simulink model "ASM_Traffic_A11"  (R2026a)
settings: Solver=ode1  StartTime=SIM.tstart.v  StopTime=SIM.tend.v  FixedStep=SIM.StepSize.v
PostLoadFcn:
  | if any(exist('dsrtsu_mdlpostloadfcn', 'file') ~= 0), dsrtsu_mdlpostloadfcn('Execute', bdroot); end
  | try, asm_mdl_postloadfcn(bdroot, 'UpdateModel', 3600); catch, disp(lasterr); end,
InitFcn:
  | , if any(exist('rtifpga_mdlclblib', 'file') ~= 0), rtifpga_mdlclblib('Init', bdroot); end,
  | , if any(exist('dsmpb_private', 'file') ~= 0), dsmpb_private('dsmpb_mdlclblib', 'Init', bdroot); end,
undefined symbols (not defined in the file): _to_, a0b2, ASM_BrakeHydraulics_DemoSystems, ASM_VehicleDynamics_DemoSystems, b98103fe8ad365046cd0, BrakeCircuit, controllerConfig, CPT, Crankshaft, DiscIntNeverNeededParam, dsmsi, FinalDriveAssembly, instance, MDL, ModeSignals, mu, Pos_BrakePedal_Maneuver, rad, RefSignals, s_to_rpm, SIM, SoftECU, Suspension, Tire, Transmission
libraries: ASM_Traffic_lib x135, simulink x98, ASM_Utils_lib x77, ASM_VehicleDynamics_lib x70, ASM_Environment_lib x22, dsmpblib x20, dsmsilib x15, MDLD_Utils_lib x10, ASM_BrakeHydraulics_lib x3, sl_discontinuities x2
(part 16 of 63)

== system ASM_Traffic_A11/VehicleDynamics/Plant/Sw_Plant_Signals ==
  PlantModel_Signals : Inport
  ExternalPlant_Signals : Inport  Port=2
  Angle_Gamma_FL_Wheel[deg] : Subsystem
  Bus Creator : BusCreator  Inputs=3
  Bus Creator1 : BusCreator  Inputs=2
  Bus Creator2 : BusCreator  Inputs=1
  Bus Creator3 : BusCreator  Inputs=2
  Bus Selector : BusSelector  OutputSignals=Steering.Displ_Steering[m],Steering.Displ_Steering_dt[m|s],RollerDyno.Angle_Gamma_FL_Wheel[deg],RollerDyno.omega_Wheel[rad|s]
  Bus Selector1 : BusSelector  OutputSignals=ExternalPlant.EPSMotor.Angle_EPSMotor[rad],ExternalPlant.EPSMotor.Angle_dt_EPSMotor[rad|s],ExternalPlant.Steering.Displ_Steering[m],ExternalPlant.Steering.Displ_Steering_dt[m|s],ExternalPlant.RollerDyno.Angle_Gamma_FL_Wheel[deg],ExternalPlant.RollerDyno.omega_Wheel[FL;FR;RL;RR][rad|s]
  Demux : Demux  Outputs=2
  Displ_SteeringRod[Displ;Displ_dt][m;m|s] : Subsystem
  EPSMotorStates_External[Angle;Angle_dt][rad;rad|s] : Subsystem
  EPS_External[Angle;Angle_dt][rad;rad|s]1 : Constant  Value=[0;0]
  Mux1 : Mux  Inputs=2
  Mux2 : Mux  Inputs=2
  Mux3 : Mux  Inputs=2
  omega_Wheel[FL;FR;RL;RR][rad|s] : Subsystem
  Plant_Signals : Outport  VectorParamsAs1DForOutWhenUnconnected=off
  wires:
  Demux/1 -> Bus Creator1/1  "Displ_Steering[m]"
  Demux/2 -> Bus Creator1/2  "Displ_Steering_dt[m|s]"
  Displ_SteeringRod[Displ;Displ_dt][m;m|s]/1(Displ_SteeringRod[Displ;Displ_dt][m;m|s]) -> Demux/1  "Displ_SteeringRod[Displ;Displ_dt][m;m|s]"
  EPS_External[Angle;Angle_dt][rad;rad|s]1/1 -> EPSMotorStates_External[Angle;Angle_dt][rad;rad|s]/1(SoftECU)
  Mux3/1 -> Displ_SteeringRod[Displ;Displ_dt][m;m|s]/1(SoftECU)
  Bus Selector/2 -> Mux3/2  "<Displ_Steering_dt[m|s]>"
  Bus Selector/1 -> Mux3/1  "<Displ_Steering[m]>"
  Mux1/1 -> EPSMotorStates_External[Angle;Angle_dt][rad;rad|s]/2(RealECU)
  Mux2/1 -> Displ_SteeringRod[Displ;Displ_dt][m;m|s]/2(RealECU)
  Bus Selector1/4 -> Mux2/2  "<Displ_Steering_dt[m|s]>"
  Bus Selector1/3 -> Mux2/1  "<Displ_Steering[m]>"
  Bus Selector1/2 -> Mux1/2  "<Angle_dt_EPSMotor[rad|s]>"
  Bus Selector1/1 -> Mux1/1  "<Angle_EPSMotor[rad]>"
  EPSMotorStates_External[Angle;Angle_dt][rad;rad|s]/1(EPSMotorStates_External[Angle;Angle_dt][rad;rad|s]) -> Bus Creator2/1  "EPSMotorStates_External[Angle;Angle_dt][rad;rad|s]"
  Bus Creator2/1 -> Bus Creator/1  "EPSMotor"
  Bus Creator1/1 -> Bus Creator/2  "Steering"
  Bus Creator/1 -> Plant_Signals/1  "ActivePlant"
  ExternalPlant_Signals/1 -> Bus Selector1/1
  PlantModel_Signals/1 -> Bus Selector/1
  Bus Selector1/5 -> Angle_Gamma_FL_Wheel[deg]/2(RealECU)  "<Angle_Gamma_FL_Wheel[deg]>"
  Bus Selector1/6 -> omega_Wheel[FL;FR;RL;RR][rad|s]/2(RealECU)  "<omega_Wheel[FL;FR;RL;RR][rad|s]>"
  omega_Wheel[FL;FR;RL;RR][rad|s]/1(omega_Wheel[FL;FR;RL;RR][rad|s]) -> Bus Creator3/2  "omega_Wheel[FL;FR;RL;RR][rad|s]"
  Angle_Gamma_FL_Wheel[deg]/1(Angle_Gamma_FL_Wheel[deg]) -> Bus Creator3/1  "Angle_Gamma_FL_Wheel[deg]"
  Bus Creator3/1 -> Bus Creator/3  "RollerDyno"
  Bus Selector/3 -> Angle_Gamma_FL_Wheel[deg]/1(SoftECU)  "<Angle_Gamma_FL_Wheel[deg]>"
  Bus Selector/4 -> omega_Wheel[FL;FR;RL;RR][rad|s]/1(SoftECU)  "<omega_Wheel[rad|s]>"

== system ASM_Traffic_A11/VehicleDynamics/Plant/UserInterface ==
  note: Vehicle Dynamics
  In : Inport
  ASMSignalBus_Plant : Subsystem
  DISP_Plant : Subsystem
  PAR_Plant : Subsystem
  Out : Outport  VectorParamsAs1DForOutWhenUnconnected=off
  wires:
  PAR_Plant/1(Out) -> Out/1
  In/1 -> ASMSignalBus_Plant/1(In), DISP_Plant/1(In)

== system ASM_Traffic_A11/VehicleDynamics/Plant/VehicleDynamics ==
  UserInterface : Inport
  Interface_In : Inport  Port=2
  Control : Inport  Port=3
  Plant_Signals : Inport  Port=4
  AERODYNAMICS : ASM_VehicleDynamics_lib/VehicleDynamics/Aerodynamics/AERODYNAMICS  Tag=ASM_SUBCOMPONENT  Map_C_x=MDL.VehicleDynamics.Aerodynamics.Map_C_x  Map_C_y=MDL.VehicleDynamics.Aerodynamics.Map_C_y  Map_C_z=MDL.VehicleDynamics.Aerodynamics.Map_C_z  Map_C_M_x=MDL.VehicleDynamics.Aerodynamics.Map_C_M_x  Map_C_M_y=MDL.VehicleDynamics.Aerodynamics.Map_C_M_y  Map_C_M_z=MDL.VehicleDynamics.Aerodynamics.Map_C_M_z  Const_A_x=MDL.VehicleDynamics.Aerodynamics.Const_A_x  Const_PosVec_VtoRefAero=MDL.VehicleDynamics.Aerodynamics.Const_PosVec_RefAero_CoorSysV  Const_Char_Length=MDL.VehicleDynamics.Aerodynamics.Const_Char_Length  Const_Dens_Air=MDL.VehicleDynamics.Aerodynamics.Const_Dens_Air  ASMProperties=struct('Name','AERODYNAMICS','Version','5.0','Library','ASM_VehicleDynamics_lib')  ASMInstanceName=aerodynamics  ASMInstanceID=1
  ASMSignalCollector : Subsystem
  Brake : Subsystem
  Bus Selector1 : BusSelector  OutputSignals=ExternalModel.Sw_Tire_Parameter_Set_CP[FL;FR;RL;RR][1|2|3|4],ExternalModel.Fric_Coeff_CP[FL;FR;RL;RR][],ExternalModel.Pos_z_CP[FL;FR;RL;RR][m],ExternalModel.UnitVec_z_CP[FL;FR;RL;RR][x;y;z],ExternalModel.Pos_Vehicle_Init_CoorSys_E[x;y;z][m],ExternalModel.Angle_Vehicle_Init_CoorSys_E[x;y;z][rad],ExternalModel.Reset_VehicleStates[0|1],ExternalModel.Keep_VehiclePosition[0|1],ExternalModel.Pos_BrakePedal[%],ExternalModel.Angle_SteeringWheel[deg],ExternalModel.v_Wind_Coor_Sys_E[x;y;z][m|s],ExternalModel.p_Ambient[Pa],ExternalModel.Sw_ParkingBrake[0Off|1On],ExternalModel.T_Ambient[degC],ExternalModel.Pos_AccPedal[%],ExternalModel.q_dt_Vehicle_Init[6x1],ExternalModel.Trq_Driver_External[Nm],ExternalModel.Sw_SteeringMode[1Angle|2Trq],ExternalModel.Sw_Steering_Mode[1Manual|2ManSched],ExternalModel.Const_Steering_Mode_Manual[1Angle|2Trq]
  Bus Selector10 : BusSelector  OutputSignals=ExternalModel.Q_Articulated_T[6x1],ExternalModel.Trq_Hitch_CoorSys_V[x;y;z][Nm],ExternalModel.M_Articulated_T[1x36]
  Bus Selector2 : BusSelector  OutputSignals=w_Rel_FL_Wheel_dDispl_SteeringRod_dt[x;y;z][rad|m],w_Rel_FR_Wheel_dDispl_SteeringRod_dt[x;y;z][rad|m]  OutputAsBus=on
  Bus Selector3 : BusSelector  OutputSignals=Pos_FL_Wheel_dDispl_SteeringRod[x;y;z][],Pos_FR_Wheel_dDispl_SteeringRod[x;y;z][]  OutputAsBus=on
  Bus Selector4 : BusSelector  OutputSignals=ECU_Steering.Trq_PowerSteering[Nm]
  Bus Selector6 : BusSelector  OutputSignals=ECU_Brake.ECU_Mode.ECU_ESP_Mode[0None|1ABS|2ESP|3ASR],ECU_Brake.Valves.Ctrl_InletValve_FL[0_1],ECU_Brake.Valves.Ctrl_InletValve_FR[0_1],ECU_Brake.Valves.Ctrl_InletValve_RL[0_1],ECU_Brake.Valves.Ctrl_InletValve_RR[0_1],ECU_Brake.Valves.Ctrl_OutletValve_FL[0_1],ECU_Brake.Valves.Ctrl_OutletValve_FR[0_1],ECU_Brake.Valves.Ctrl_OutletValve_RL[0_1],ECU_Brake.Valves.Ctrl_OutletValve_RR[0_1],ECU_Brake.Valves.Ctrl_PreChargeValve_1[0_1],ECU_Brake.Valves.Ctrl_PreChargeValve_2[0_1],ECU_Brake.Valves.Ctrl_ChangeOverValve_1[0_1],ECU_Brake.Valves.Ctrl_ChangeOverValve_2[0_1],ECU_Brake.Valves.Ctrl_HydPump[0_1],ECU_Brake.DesiredPressure.Enable_p_Brake_Desired[0|1],ECU_Brake.DesiredPressure.p_Brake_Desired[bar]  OutputAsBus=on
  Bus Selector7 : BusSelector  OutputSignals=Tire.Tire.Sw_r_Tire[1:intern;2:extern],Tire.Tire.r_Tire_extern[m],Suspension.Suspension_Init.q_dt_Wheel_Init[:],Suspension.Suspension_Init.q_Wheel_Init[:],BrakeHydraulics.Sw_DistributionPattern_[1X|2II],Suspension.Sw_Rotation[1Cardan|2ToeCamberCaster]
  Bus Selector8 : BusSelector  OutputSignals=Steering.Displ_Steering_dt[m|s],Steering.Displ_Steering[m],RollerDyno.omega_Wheel[FL;FR;RL;RR][rad|s],EPSMotor.EPSMotorStates_External[Angle;Angle_dt][rad;rad|s],RollerDyno.Angle_Gamma_FL_Wheel[deg]
  Bus Selector9 : BusSelector  OutputSignals=ExternalModel.Trq_Shaft[FL;FR;RL;RR][Nm]
  CommonVehicleParameters : Subsystem
      settings: CopyFcn=|
      | try
      |  set_param(gcb,'LinkStatus', 'none')
      | catch
      | end
      mask Display: disp('Common vehicle parameters')
  Constant : Constant  Value=0
  DerivativeAddition : Subsystem
  Exchangeable_Plant_Signals : Subsystem
  Goto Tag Visibility : GotoTagVisibility  GotoTag=ASMBUS_VehicleDynamics_Tire
  Goto Tag Visibility1 : GotoTagVisibility  GotoTag=ASMBUS_VehicleDynamics_Aerodynamics
  Goto Tag Visibility10 : GotoTagVisibility  GotoTag=TAG_VehicleDynamics_Inertia_y_RL_Wheel
  Goto Tag Visibility11 : GotoTagVisibility  GotoTag=TAG_VehicleDynamics_Inertia_y_RR_Wheel
  Goto Tag Visibility12 : GotoTagVisibility  GotoTag=TAG_VehicleDynamics_Coef_DynamicBrakeTrq
  Goto Tag Visibility13 : GotoTagVisibility  GotoTag=TAG_VehicleDynamics_m_RR_Wheel
  Goto Tag Visibility14 : GotoTagVisibility  GotoTag=TAG_VehicleDynamics_Inertia_FL_Wheel
  Goto Tag Visibility15 : GotoTagVisibility  GotoTag=TAG_VehicleDynamics_Inertia_FR_Wheel
  Goto Tag Visibility16 : GotoTagVisibility  GotoTag=TAG_VehicleDynamics_Inertia_RL_Wheel
  Goto Tag Visibility17 : GotoTagVisibility  GotoTag=TAG_VehicleDynamics_Inertia_RR_Wheel
  Goto Tag Visibility18 : GotoTagVisibility  GotoTag=TAG_VehicleDynamics_Inertia_y_FL_Wheel
  Goto Tag Visibility19 : GotoTagVisibility  GotoTag=TAG_VehicleDynamics_Inertia_y_FR_Wheel
  Goto Tag Visibility2 : GotoTagVisibility  GotoTag=ASMBUS_VehicleDynamics_VehicleMovement
  Goto Tag Visibility20 : GotoTagVisibility  GotoTag=ASMBUS_VehicleDynamics_Steering_Rod_Back_Calc
  Goto Tag Visibility3 : GotoTagVisibility  GotoTag=ASMBUS_VehicleDynamics_WheelSpeed
  Goto Tag Visibility4 : GotoTagVisibility  GotoTag=ASMBUS_VehicleDynamics_Suspension
  Goto Tag Visibility5 : GotoTagVisibility  GotoTag=ASMBUS_VehicleDynamics_Brake
  Goto Tag Visibility6 : GotoTagVisibility  GotoTag=ASMBUS_VehicleDynamics_Steering
  Goto Tag Visibility7 : GotoTagVisibility  GotoTag=TAG_VehicleDynamics_m_FL_Wheel
  Goto Tag Visibility8 : GotoTagVisibility  GotoTag=TAG_VehicleDynamics_m_FR_Wheel
  Goto Tag Visibility9 : GotoTagVisibility  GotoTag=TAG_VehicleDynamics_m_RL_Wheel
  Hitch_Vehicle : Subsystem
      settings: CopyFcn=|
      | try
      |  set_param(gcb,'LinkStatus', 'none')
      | catch
      | end
  ModelDesk_MC_ID_VehicleDynamics : ASM_Utils_lib/ModelDeskInterface/ModelDesk_MC  Tag=ASM_MAINCOMPONENT  Editable=off  MainComponent=VehicleDynamics
  Multiport Switch : MultiPortSwitch  Inputs=2  SaturateOnIntegerOverflow=off  InputSameDT=off
  OR : Subsystem
  STEERING_3DOF_VARIABLE_RATIO : ASM_VehicleDynamics_lib/VehicleDynamics/Steering/STEERING_3DOF_VARIABLE_RATIO  Tag=ASM_SUBCOMPONENT  SW_EPSLocation=MDL.VehicleDynamics.Steering3DOF.SW_EPSLocation  SW_EPSSimulation=MDL.VehicleDynamics.Steering3DOF.SW_EPSSimulation  SW_ExternalEPSOutput=MDL.VehicleDynamics.Steering3DOF.SW_ExternalEPSOutput  SW_LocationColumnStiffness=MDL.VehicleDynamics.Steering3DOF.SW_LocationColumnStiffness  SW_DriverHand=MDL.VehicleDynamics.Steering3DOF.SW_DriverHand  Map_i_Steering=MDL.VehicleDynamics.Steering3DOF.Map_i_Steering  Const_i_EPSSteeringColumn=MDL.VehicleDynamics.Steering3DOF.Const_i_EPSSteeringColumn  Const_i_EPSSteeringRod=MDL.VehicleDynamics.Steering3DOF.Const_i_EPSSteeringRod  Const_Angle_Max_SteeringWheel=MDL.VehicleDynamics.Steering3DOF.Const_Angle_Max_SteeringWheel  Const_CardanAngle_UpperJoint=MDL.VehicleDynamics.Steering3DOF.Const_CardanAngle_UpperJoint  Const_CardanAngle_LowerJoint=MDL.VehicleDynamics.Steering3DOF.Const_CardanAngle_LowerJoint  Const_AngleOffsetCardanJoints=MDL.VehicleDynamics.Steering3DOF.Const_InitialAngle_LowerCardanJoint  Const_InitialAngle_UpperCardanJoint=MDL.VehicleDynamics.Steering3DOF.Const_InitialAngle_UpperCardanJoint  Const_MaxTorque_Driver=MDL.VehicleDynamics.Steering3DOF.Const_MaxTorque_Driver  Const_Inertia_SteeringWheel=MDL.VehicleDynamics.Steering3DOF.Const_Inertia_SteeringWheel  Const_Inertia_LowerSteeringColumn=MDL.VehicleDynamics.Steering3DOF.Const_Inertia_LowerSteeringColumn  SW_SteeringColumn_Stiffness=MDL.VehicleDynamics.Steering3DOF.SW_SteeringColumn_Stiffness  Map_TrqSpring_SteeringColumn=MDL.VehicleDynamics.Steering3DOF.Map_TrqSpring_SteeringColumn  Const_Stiffness_SteeringColumn=MDL.VehicleDynamics.Steering3DOF.Const_Stiffness_SteeringColumn  Const_Damping_SteeringColumn=MDL.VehicleDynamics.Steering3DOF.Const_Damping_SteeringColumn  Const_Time_SteeringWheel=MDL.VehicleDynamics.Steering3DOF.Const_Time_SteeringWheel  Const_Stiffness_DriverHand=MDL.VehicleDynamics.Steering3DOF.Const_Stiffness_DriverHand  Const_Damping_DriverHand=MDL.VehicleDynamics.Steering3DOF.Const_Damping_DriverHand  Const_Inertia_EPS=MDL.VehicleDynamics.Steering3DOF.Const_Inertia_EPS  Const_Stiffness_EPS=MDL.VehicleDynamics.Steering3DOF.Const_Stiffness_EPS  Const_Damping_EPS=MDL.VehicleDynamics.Steering3DOF.Const_Damping_EPS  Const_Damping_LowerSteeringColumn=MDL.VehicleDynamics.Steering3DOF.Const_Damping_LowerSteeringColumn  SW_SF_SteeringWheel=MDL.VehicleDynamics.Steering3DOF.SpringFriction.SW_SF_SteeringWheel  Const_Stiffness_SF_SteeringWheel=MDL.VehicleDynamics.Steering3DOF.SpringFriction.Const_Stiffness_SF_SteeringWheel  Const_LimitingTorque_SF_SteeringWheel=MDL.VehicleDynamics.Steering3DOF.SpringFriction.Const_LimitingTorque_SF_SteeringWheel  SW_ESF_SteeringWheel=MDL.VehicleDynamics.Steering3DOF.ExponentialSpringFriction.SW_ESF_SteeringWheel  Const_Stiffness_ESF_SteeringWheel=MDL.VehicleDynamics.Steering3DOF.ExponentialSpringFriction.Const_Stiffness_ESF_SteeringWheel  Const_LimitingTorque_ESF_SteeringWheel=MDL.VehicleDynamics.Steering3DOF.ExponentialSpringFriction.Const_LimitingTorque_ESF_SteeringWheel  SW_CF_SteeringRod=MDL.VehicleDynamics.Steering3DOF.CoulombFriction.SW_CF_SteeringRod  Const_LimitingForce_CF_SteeringRod=MDL.VehicleDynamics.Steering3DOF.CoulombFriction.Const_LimitingForce_CF_SteeringRod  Const_Damping_CF_SteeringRod=MDL.VehicleDynamics.Steering3DOF.CoulombFriction.Const_Damping_CF_SteeringRod  SW_MF_SteeringRod=MDL.VehicleDynamics.Steering3DOF.MaxwellFriction.SW_MF_SteeringRod  Const_Stiffness_MF_SteeringRod=MDL.VehicleDynamics.Steering3DOF.MaxwellFriction.Const_Stiffness_MF_SteeringRod  Const_LimitingForce_MF_SteeringRod=MDL.VehicleDynamics.Steering3DOF.MaxwellFriction.Const_LimitingForce_MF_SteeringRod  Const_Damping_MF_SteeringRod=MDL.VehicleDynamics.Steering3DOF.MaxwellFriction.Const_Damping_MF_SteeringRod  SW_SF_SteeringRod=MDL.VehicleDynamics.Steering3DOF.SpringFriction.SW_SF_SteeringRod  Const_Stiffness_SF_SteeringRod=MDL.VehicleDynamics.Steering3DOF.SpringFriction.Const_Stiffness_SF_SteeringRod  Const_LimitingForce_SF_SteeringRod=MDL.VehicleDynamics.Steering3DOF.SpringFriction.Const_LimitingForce_SF_SteeringRod  SW_ESF_SteeringRod=MDL.VehicleDynamics.Steering3DOF.ExponentialSpringFriction.SW_ESF_SteeringRod  Const_Stiffness_ESF_SteeringRod=MDL.VehicleDynamics.Steering3DOF.ExponentialSpringFriction.Const_Stiffness_ESF_SteeringRod  Const_LimitingForce_ESF_SteeringRod=MDL.VehicleDynamics.Steering3DOF.ExponentialSpringFriction.Const_LimitingForce_ESF_SteeringRod  StepSize=SIM.StepSize  ASMProperties=struct('Name','STEERING_3DOF_VARIABLE_RATIO','Version','10.0','Library','ASM_VehicleDynamics_lib')  ASMInstanceName=steering_3dof_variable_ratio  ASMInstanceID=1
  STEERING_ROD_BACK_CALC : ASM_VehicleDynamics_lib/VehicleDynamics/STEERING_ROD_BACK_CALC  Tag=ASM_SUBCOMPONENT  Map_Displ_SteeringRod=MDL.VehicleDynamics.SteeringRodBackCalc.Map_Displ_SteeringRod  Sw_Backward_SteeringRod_Calc=MDL.VehicleDynamics.SteeringRodBackCalc.Sw_Backward_SteeringRod_Calc  Const_NaturalFrequency_Displ_SteeringRod=MDL.VehicleDynamics.SteeringRodBackCalc.Const_NaturalFrequency_Displ_SteeringRod  ASMProperties=struct('Name','STEERING_ROD_BACK_CALC','Version','1.0','Library','ASM_VehicleDynamics_lib')  ASMInstanceName=steering_rod_back_calc  ASMInstanceID=1
  SignalSpecification : SignalSpecification  Dimensions=4
  Suspension : Subsystem
  Terminator{,1..3} (4 alike) : Terminator
  Tire : Subsystem
  TireMapping_CP : Subsystem
      mask Display: disp('');
  VehicleInits : Subsystem
  VehicleMovement : Subsystem
  WHEEL_SPEED : ASM_VehicleDynamics_lib/VehicleDynamics/WheelSpeed/WHEEL_SPEED  Tag=ASM_SUBCOMPONENT  StepSize=SIM.StepSize  ASMProperties=struct('Name','WHEEL_SPEED','Version','11.0','Library','ASM_VehicleDynamics_lib')  ASMInstanceName=wheel_speed  ASMInstanceID=1
  "[1x36]to[6x6]" : Reshape  OutputDimensionality=Customize  OutputDimensions=[6,6]
  avoid_incomplete_trace2source : Subsystem
  avoid_incomplete_trace2source1 : Subsystem
  avoid_incomplete_trace2source2 : Subsystem
  ASMSignalBus : Outport  VectorParamsAs1DForOutWhenUnconnected=off
  PlantModel_Signals : Outport  Port=2  VectorParamsAs1DForOutWhenUnconnected=off
  tag scope: ASMBUS_VehicleDynamics_Aerodynamics=scoped, ASMBUS_VehicleDynamics_Brake=scoped, ASMBUS_VehicleDynamics_Steering=scoped, ASMBUS_VehicleDynamics_Steering_Rod_Back_Calc=scoped, ASMBUS_VehicleDynamics_Suspension=scoped, ASMBUS_VehicleDynamics_Tire=scoped, ASMBUS_VehicleDynamics_VehicleMovement=scoped, ASMBUS_VehicleDynamics_WheelSpeed=scoped
  wires:
  avoid_incomplete_trace2source2/1(Out1) -> WHEEL_SPEED/7
  Bus Selector8/3 -> avoid_incomplete_trace2source2/1(In1)  "<omega_Wheel[FL;FR;RL;RR][rad|s]>"
  avoid_incomplete_trace2source1/1(Out1) -> WHEEL_SPEED/5
  avoid_incomplete_trace2source/1(Out1) -> WHEEL_SPEED/1
  Tire/5(Trq_Tire_Wheel[FL,FR,RL,RR][Nm]) -> avoid_incomplete_trace2source/1(In1)
  Bus Selector8/5 -> STEERING_ROD_BACK_CALC/1  "<Angle_Gamma_FL_Wheel[deg]>"
  Interface_In/1 -> Bus Selector10/1, Bus Selector1/1, Bus Selector9/1
  Brake/1(ASMSignalBus) -> [ASMBUS_VehicleDynamics_Brake]
  AERODYNAMICS/1 -> [ASMBUS_VehicleDynamics_Aerodynamics]
  WHEEL_SPEED/1 -> [ASMBUS_VehicleDynamics_WheelSpeed]
  WHEEL_SPEED/3 -> VehicleMovement/6(w_Wheel[FL,FR,RL,RR][x;y;z][rad|s])
  Tire/3(Trq_Tire_CoorSys_V[FL,FR,RL,RR][x;y;z][Nm]) -> VehicleMovement/4(Trq_Tire_CoorSys_V[FL,FR,RL,RR][x;y;z][Nm]), STEERING_3DOF_VARIABLE_RATIO/4, Suspension/4(Trq_Tire[FL;FR;RL;RR][x;y;z][Nm])
  STEERING_3DOF_VARIABLE_RATIO/1 -> [ASMBUS_VehicleDynamics_Steering]
  Tire/2(F_Tire_CoorSys_V[FL,FR,RL,RR][x;y;z][N]) -> STEERING_3DOF_VARIABLE_RATIO/3, Suspension/3(F_Tire[FL;FR;RL;RR][x;y;z][N]), VehicleMovement/3(F_Tire_CoorSys_V[FL,FR,RL,RR][x;y;z][N])
  VehicleMovement/4(Pos_Wheels_CoorSys_E[FL,FR,RL,RR][x;y;z][m]) -> Tire/3(Pos_Wheels_CoorSys_E[FL,FR,RL,RR][x,y,z][m])
  VehicleMovement/5(v_Abs_WheelBody_CoorSys_V[FL,FR,RL,RR][x y z][m|s]) -> Tire/4(v_Abs_WheelBody_CoorSys_V[FL,FR,RL,RR][x;y;z][m|s])
  VehicleMovement/6(w_Abs_Wheel_CoorSys_V[FL,FR,RL,RR][x,y,z][rad|s]) -> Tire/5(w_Abs_Wheel_CoorSys_V[FL,FR,RL,RR][x,y,z][rad|s])
  VehicleMovement/3(RotationMatrix_V_to_E_T[3x3]) -> Tire/2(RotationMatrix_V_to_E_T[3x3]), AERODYNAMICS/1
  AERODYNAMICS/2 -> VehicleMovement/2(Trq_Aero_CoorSys_V[x;y;z][Nm])
  AERODYNAMICS/3 -> VehicleMovement/1(F_Aero_CoorSys_V[x;y;z][N])
  VehicleMovement/1(ASMSignalBus) -> [ASMBUS_VehicleDynamics_VehicleMovement]
  VehicleMovement/2(v_Abs_Vehicle_CoG[x;y;z][m|s]) -> AERODYNAMICS/2
  Brake/2(Trq_Brake[FL,FR,RL,RR][Nm]) -> WHEEL_SPEED/3
  Bus Selector1/7 -> Brake/1(Reset[]), STEERING_ROD_BACK_CALC/4, STEERING_3DOF_VARIABLE_RATIO/7, OR/2(In2), VehicleMovement/14(Reset[]), Suspension/6(Reset[]), avoid_incomplete_trace2source1/1(In1)  "<Reset_VehicleStates[0|1]>"
  Bus Selector1/9 -> Brake/2(Pos_BrakePedal[%])  "<Pos_BrakePedal[%]>"
  Bus Selector1/11 -> AERODYNAMICS/3  "<v_Wind_Coor_Sys_E[x;y;z][m|s]>"
  Suspension/1(ASMSignalBus) -> [ASMBUS_VehicleDynamics_Suspension]
  VehicleMovement/8(Trq_Gyroscopic[FL,FR,RL,RR][x;y;z][Nm]) -> STEERING_3DOF_VARIABLE_RATIO/9
  VehicleMovement/7(F_Gyroscopic[FL,FR,RL,RR][x;y;z][N]) -> STEERING_3DOF_VARIABLE_RATIO/8
  VehicleMovement/9(F_Gravitational[FL,FR,RL,RR][x;y;z][N]) -> STEERING_3DOF_VARIABLE_RATIO/10
  Suspension/10(UnitVec_y_Wheel_CoorSys_V[FL,FR,RL,RR][x;y;z]) -> Tire/1(UnitVec_y_Wheel_CoorSys_V[FL,FR,RL,RR][x;y;z]), WHEEL_SPEED/4
  Bus Selector6/1 -> Brake/3(IO_Signals)
  Bus Selector1/6 -> VehicleMovement/13(Angle_V_Init_CoorSys_E[x;y;z][rad])  "<Angle_Vehicle_Init_CoorSys_E[x;y;z][rad]>"
  Bus Selector1/5 -> VehicleMovement/12(Pos_Vehicle_Init_CoorSys_E[x;y;z][m])  "<Pos_Vehicle_Init_CoorSys_E[x;y;z][m]>"
  Tire/1(ASMSignalBus) -> [ASMBUS_VehicleDynamics_Tire]
  Tire/4(Stiffness_z_Tire[FL,FR,RL,RR][N|m]) -> VehicleMovement/5(Stiffness_z_Tire[FL,FR,RL,RR][N|m])
  Bus Selector9/1 -> SignalSpecification/1  "<Trq_Shaft[FL;FR;RL;RR][Nm]>"
  WHEEL_SPEED/4 -> Exchangeable_Plant_Signals/1(omega_Wheel[rad|s]), Tire/11(omega_Wheel[FL,FR,RL,RR][rad|s])
  WHEEL_SPEED/2 -> STEERING_3DOF_VARIABLE_RATIO/5, VehicleMovement/7(Trq_Shaft_CoorSys_V[FL,FR,RL,RR][x;y;z][Nm])
  Suspension/9(gF_Susp[q1_Front;q2_Front;q1_Rear;q2_Rear][]) -> VehicleMovement/8(gF_Susp[q1_Front;q2_Front;q1_Rear;q2_Rear][])
  Suspension/8(Pos_Wheels[FL,FR,RL,RR][x;y;z][m]) -> VehicleMovement/9(Pos_Wheel[FL,FR,RL,RR][x;y;z][m])
  Suspension/7(w_Rel_WheelBody[FL,FR,RL,RR][x;y;z][x;y;z][rad|s]) -> VehicleMovement/10(w_Rel_WheelBody[FL,FR,RL,RR][x y z][rad|s])
  Suspension/6(v_Rel_WheelBody[FL,FR,RL,RR][x;y;z][m|s]) -> VehicleMovement/11(v_Rel_WheelBody[FL,FR,RL,RR][x;y;z][m|s])
  VehicleMovement/10(q_Wheel_dt[q1_Front;q2_Front;q1_Rear;q2_Rear][]) -> Suspension/2(q_Wheel_dt[q1_Front;q2_Front;q1_Rear;q2_Rear][])
  VehicleMovement/11(q_Wheel[q1_Front;q2_Front;q1_Rear;q2_Rear][]) -> Suspension/1(q_Wheel[q1_Front;q2_Front;q1_Rear;q2_Rear][])
  Suspension/2(SuspensionKinematicRelations_Front) -> VehicleMovement/19(SuspensionKinematicsRelations_Front), Bus Selector3/1, Bus Selector2/1
  Suspension/3(SuspensionKinematicRelations_Rear) -> VehicleMovement/18(SuspensionKinematicsRelations_Rear)
  Suspension/4(gFront_dq_Front_dt[2x2][]) -> VehicleMovement/17(gFront_dq_Front_dt[2x2][])
  Suspension/5(gRear_dq_Rear_dt[2x2][]) -> VehicleMovement/16(gRear_dq_Rear_dt[2x2][])
  Bus Selector1/10 -> DerivativeAddition/1(Angle_SteeringWheel_Driver[deg])  "<Angle_SteeringWheel[deg]>"
  Bus Selector1/12 -> Brake/4(p_Ambient[Pa])  "<p_Ambient[Pa]>"
  SignalSpecification/1 -> WHEEL_SPEED/2
  Bus Selector1/13 -> Brake/5(Sw_ParkingBrake[0Off|1On])  "<Sw_ParkingBrake[0Off|1On]>"
  Hitch_Vehicle/1(F_External_CoorSys_V[x;y;z][N]) -> VehicleMovement/20(F_External_CoorSys_V[x,y,z][N])
  Hitch_Vehicle/2(Trq_External_CoorSys_V[x;y;z][Nm]) -> VehicleMovement/21(Trq_External_CoorSys_V[x,y,z][Nm])
  Hitch_Vehicle/3(Stabilization_F_External[3x6]) -> VehicleMovement/22(Stabilization_F_External[3X6])
  Hitch_Vehicle/4(Stabilization_Trq_External[3x6]) -> VehicleMovement/23(Stabilization_Trq_External[3X6])
  STEERING_3DOF_VARIABLE_RATIO/4 -> Terminator/1
  Bus Selector1/14 -> Brake/6(T_Ambient[degC])  "<T_Ambient[degC]>"
  Bus Selector1/15 -> Brake/7(Pos_AccPedal[%])  "<Pos_AccPedal[%]>"
  Bus Selector1/8 -> VehicleMovement/15(KeepVehiclePosition[0|1]), OR/1(In1)  "<Keep_VehiclePosition[0|1]>"
  OR/1(Out) -> Tire/10(Reset[])
  VehicleInits/1(omega_Wheel_Init[:][rad|s]) -> WHEEL_SPEED/6
  Bus Selector1/1 -> TireMapping_CP/1(Sw_Tire_Parameter_Set_CP[:][1|2|3|4])  "<Sw_Tire_Parameter_Set_CP[FL;FR;RL;RR][1|2|3|4]>"
  Bus Selector1/16 -> VehicleInits/1(q_dt_Vehicle_Init[6x1])  "<q_dt_Vehicle_Init[6x1]>"
  VehicleInits/3(q_Wheel_Init[:]) -> VehicleMovement/25(q_Wheel_Init[:])
  VehicleInits/2(q_dt_Init[:]) -> VehicleMovement/24(q_dt_Init[:])
  DerivativeAddition/1(SteeringWheel_Driver[Angle;Angle_dt][deg;deg|s]) -> STEERING_3DOF_VARIABLE_RATIO/6
  Bus Selector2/1 -> STEERING_3DOF_VARIABLE_RATIO/1
  Bus Selector3/1 -> STEERING_3DOF_VARIABLE_RATIO/2
  Bus Selector1/17 -> STEERING_3DOF_VARIABLE_RATIO/12  "<Trq_Driver_External[Nm]>"
  Bus Selector1/18 -> Multiport Switch/3  "<Sw_SteeringMode[1Angle|2Trq]>"
  Constant/1 -> Suspension/5(AirSuspensionSignals_In)
  Suspension/11(AirSuspensionSignals_Out) -> Terminator3/1
  Bus Selector1/19 -> Multiport Switch/1  "<Sw_Steering_Mode[1Manual|2ManSched]>"
  Bus Selector1/20 -> Multiport Switch/2  "<Const_Steering_Mode_Manual[1Angle|2Trq]>"
  Multiport Switch/1 -> STEERING_3DOF_VARIABLE_RATIO/13
  Control/1 -> Bus Selector6/1, Bus Selector4/1
  Bus Selector4/1 -> STEERING_3DOF_VARIABLE_RATIO/14  "<Trq_PowerSteering[Nm]>"
  Plant_Signals/1 -> Bus Selector8/1
  ASMSignalCollector/1(ASMSignalBus) -> ASMSignalBus/1
  UserInterface/1 -> Bus Selector7/1
  Bus Selector8/1 -> Suspension/8(Displ_SteeringRod_dt[m|s])  "<Displ_Steering_dt[m|s]>"
  Bus Selector8/2 -> Suspension/9(Displ_SteeringRod[m])  "<Displ_Steering[m]>"
  Bus Selector8/4 -> STEERING_3DOF_VARIABLE_RATIO/11  "<EPSMotorStates_External[Angle;Angle_dt][rad;rad|s]>"
  Bus Selector7/6 -> Suspension/7(Sw_Rotation[1Cardan|2ToeCamberCaster])  "<Sw_Rotation[1Cardan|2ToeCamberCaster]>"
  Bus Selector7/1 -> Tire/12(Sw_r_Tire[1:intern;2:extern])  "<Sw_r_Tire[1:intern;2:extern]>"
  Bus Selector7/3 -> VehicleInits/2(q_dt_Wheel_Init[:])  "<q_dt_Wheel_Init[:]>"
  Bus Selector7/4 -> VehicleInits/3(q_Wheel_Init_In[:])  "<q_Wheel_Init[:]>"
  Bus Selector7/5 -> Brake/8(Sw_DistributionPattern[1X|2II])  "<Sw_DistributionPattern_[1X|2II]>"
  STEERING_3DOF_VARIABLE_RATIO/3 -> STEERING_ROD_BACK_CALC/3
  Exchangeable_Plant_Signals/1(Out) -> PlantModel_Signals/1
  STEERING_3DOF_VARIABLE_RATIO/2 -> STEERING_ROD_BACK_CALC/2
  Bus Selector7/2 -> Tire/13(r_Tire_extern[m])  "<r_Tire_extern[m]>"
  Bus Selector10/3 -> "[1x36]to[6x6]"/1  "<M_Articulated_T[1x36]>"
  "[1x36]to[6x6]"/1 -> Hitch_Vehicle/3(M_Articulated_T[6x6])
  Bus Selector10/2 -> Hitch_Vehicle/2(Trq_Hitch_CoorSys_V[x;y;z][Nm])  "<Trq_Hitch_CoorSys_V[x;y;z][Nm]>"
  Bus Selector10/1 -> Hitch_Vehicle/1(Q_Articulated_T[6x1])  "<Q_Articulated_T[6x1]>"
  TireMapping_CP/1(Sw_Tire_Parameter_Set_CP_Veh[FL;FR;RL;RR][1|2|3|4]) -> Tire/6(Sw_Tire_Parameter_Set[FL,FR,RL,RR][1|2|3|4])
  Bus Selector1/2 -> TireMapping_CP/2(Fric_Coeff_CP[:][])  "<Fric_Coeff_CP[FL;FR;RL;RR][]>"
  Bus Selector1/3 -> TireMapping_CP/3(Pos_z_CP[:][m])  "<Pos_z_CP[FL;FR;RL;RR][m]>"
  Bus Selector1/4 -> TireMapping_CP/4(UnitVec_z_CP[:][x;y;z])  "<UnitVec_z_CP[FL;FR;RL;RR][x;y;z]>"
  TireMapping_CP/2(Fric_Coeff_CP_Veh[FL;FR;RL;RR][]) -> Tire/7(Coef_Fric_Road[FL,FR,RL,RR][])
  TireMapping_CP/3(Pos_z_CP_Veh[FL;FR;RL;RR][m]) -> Tire/8(" Pos_z_CP_CoorSys_E[FL,FR,RL,RR][m]")
  TireMapping_CP/4(UnitVec_z_CP_Veh[FL;FR;RL;RR][x;y;z]) -> Tire/9(UnitVec_z_CP_CoorSys_E[FL,FR,RL,RR][x;y;z])
  STEERING_ROD_BACK_CALC/1 -> [ASMBUS_VehicleDynamics_Steering_Rod_Back_Calc]
  STEERING_ROD_BACK_CALC/2 -> Terminator1/1
  STEERING_ROD_BACK_CALC/3 -> Terminator2/1

== system ASM_Traffic_A11/VehicleDynamics/SignalInterface/ASMSignalInterface ==
  ASMSignalBus : Inport
  Enable : EnablePort
  signal_structure : Subsystem
  wires:
  ASMSignalBus/1 -> signal_structure/1(ASMSignalBus)

== system ASM_Traffic_A11/VehicleDynamics/SignalInterface/ExternalOutports ==
  In1 : Inport
  Enable : EnablePort
  Select_Outport_Signals : Subsystem
  VehicleDynamics : dsmpblib/Data Outport  Tag=ASM_MPB  Priority=-10000
      settings: SourceProductName=dSPACE Model Interface Package for Simulink (MIPS)
  wires:
  In1/1 -> Select_Outport_Signals/1(ASMSignalBus)
  Select_Outport_Signals/7(Aerodynamics) -> VehicleDynamics/7
  Select_Outport_Signals/6(Suspension) -> VehicleDynamics/6
  Select_Outport_Signals/5(Steering) -> VehicleDynamics/5
  Select_Outport_Signals/4(Brake) -> VehicleDynamics/4
  Select_Outport_Signals/3(WheelSpeed) -> VehicleDynamics/3
  Select_Outport_Signals/2(Tire) -> VehicleDynamics/2
  Select_Outport_Signals/1(Vehicle_Movement) -> VehicleDynamics/1

== system ASM_Traffic_A11/AnimationInterface/ANIMATION_INTERFACE/ASM_Vehicle/Chassis ==
  VehicleDynamics_Animation : Inport
  Bus Selector1 : BusSelector  OutputSignals=Pos_Vehicle_CoorSys_E[x;y;z][m],Angle_Vehicle_CoorSys_E[x;y;z][deg]
  Bus to Vector : BusToVector
  Bus to Vector1 : BusToVector
  Rotation_Chassis : Selector  InputPortWidth=3  IndexOptions=Index vector (dialog)  Indices=[3 2 1]  OutputSizes=1
  Translation : Outport
  Rotation : Outport  Port=2
  wires:
  Bus Selector1/2 -> Bus to Vector1/1  "<Angle_Vehicle_CoorSys_E[x;y;z][deg]>"
  Bus Selector1/1 -> Bus to Vector/1  "<Pos_Vehicle_CoorSys_E[x;y;z][m]>"
  VehicleDynamics_Animation/1 -> Bus Selector1/1
  Bus to Vector/1 -> Translation/1
  Rotation_Chassis/1 -> Rotation/1
  Bus to Vector1/1 -> Rotation_Chassis/1

== system ASM_Traffic_A11/AnimationInterface/ANIMATION_INTERFACE/ASM_Vehicle/Steering_Wheel ==
  VehicleDynamics_Animation : Inport
  Angle_inclination[deg] : Constant  Value=205
  Bus Selector1 : BusSelector  OutputSignals=Angle_SteeringWheel[deg]
  Mux1 : Mux  Inputs=3
  Pos_SteeringWheel[m] : Constant  Value=[-1.3, 0.35, 0.53]
  const : Constant  Value=0
  Translation : Outport
  Rotation : Outport  Port=2
  wires:
  const/1 -> Mux1/1
  Angle_inclination[deg]/1 -> Mux1/2
  Bus Selector1/1 -> Mux1/3  "<Angle_SteeringWheel[deg]>"
  VehicleDynamics_Animation/1 -> Bus Selector1/1
  Pos_SteeringWheel[m]/1 -> Translation/1
  Mux1/1 -> Rotation/1

== system ASM_Traffic_A11/AnimationInterface/ANIMATION_INTERFACE/ASM_Vehicle/TireForceLeftFront ==
  VehicleDynamics_Animation : Inport
  Bus Selector1 : BusSelector  OutputSignals=Pos_FL_Wheel[x;y;z][m],r_Dyn_FL_Tire[m],F_FL_Tire_CoorSys_V[x;y;z][N]
  Demux : Demux  Outputs=3
  Demux2 : Demux  Outputs=3
      settings: DisplayOption=none
  Mux{,1..3} (4 alike) : Mux  Inputs=3
  Product2 : Product  SaturateOnIntegerOverflow=on  OutDataTypeStr=Inherit: Same as first input
  Sum : Sum  Inputs=+-+  InputSameDT=on  SaturateOnIntegerOverflow=on  OutDataTypeStr=Inherit: Same as first input
  Sum1 : Sum  InputSameDT=on  SaturateOnIntegerOverflow=on  OutDataTypeStr=Inherit: Same as first input
  Translation_L : Outport  VectorParamsAs1DForOutWhenUnconnected=off
  Scaling_L_x : Outport  Port=2  VectorParamsAs1DForOutWhenUnconnected=off
  Scaling_L_y : Outport  Port=3  VectorParamsAs1DForOutWhenUnconnected=off
  Scaling_L_z : Outport  Port=4  VectorParamsAs1DForOutWhenUnconnected=off
  wires:
  Demux/2 -> Mux1/3
  Demux/3 -> Mux2/3
  Sum1/1 -> Mux/2
  [Pos_y_Offset_Arrow] -> Sum1/1
  Mux3/1 -> Scaling_L_x/1
  Demux/1 -> Mux3/3
  Mux1/1 -> Scaling_L_y/1
  Mux2/1 -> Scaling_L_z/1
  [Scaling_Fxy_Arrow] -> Mux2/2, Mux2/1, Mux1/2, Mux1/1, Mux3/2, Mux3/1
  Product2/1 -> Demux/1
  VehicleDynamics_Animation/1 -> Bus Selector1/1
  Bus Selector1/2 -> Sum/2  "<r_Dyn_FL_Tire[m]>"
  Sum/1 -> Mux/3
  Demux2/3 -> Sum/1
  Demux2/2 -> Sum1/2
  Demux2/1 -> Mux/1
  Bus Selector1/1 -> Demux2/1  "<Pos_FL_Wheel[x;y;z][m]>"
  Bus Selector1/3 -> Product2/1  "<F_FL_Tire_CoorSys_V[x;y;z][N]>"
  [Scaling_F_Tire] -> Product2/2
  [Pos_z_Offset_Arrow] -> Sum/3
  Mux/1 -> Translation_L/1

== system ASM_Traffic_A11/AnimationInterface/ANIMATION_INTERFACE/ASM_Vehicle/TireForceLeftRear ==
  VehicleDynamics_Animation : Inport
  Bus Selector1 : BusSelector  OutputSignals=Pos_RL_Wheel[x;y;z][m],r_Dyn_RL_Tire[m],F_RL_Tire_CoorSys_V[x;y;z][N]
  Demux : Demux  Outputs=3
  Demux2 : Demux  Outputs=3
      settings: DisplayOption=none
  Mux{,1..3} (4 alike) : Mux  Inputs=3
  Product2 : Product  SaturateOnIntegerOverflow=on  OutDataTypeStr=Inherit: Same as first input
  Sum : Sum  Inputs=+-+  InputSameDT=on  SaturateOnIntegerOverflow=on  OutDataTypeStr=Inherit: Same as first input
  Sum1 : Sum  InputSameDT=on  SaturateOnIntegerOverflow=on  OutDataTypeStr=Inherit: Same as first input
  Translation_L : Outport  VectorParamsAs1DForOutWhenUnconnected=off
  Scaling_L_x : Outport  Port=2  VectorParamsAs1DForOutWhenUnconnected=off
  Scaling_L_y : Outport  Port=3  VectorParamsAs1DForOutWhenUnconnected=off
  Scaling_L_z : Outport  Port=4  VectorParamsAs1DForOutWhenUnconnected=off
  wires:
  Demux/2 -> Mux1/3
  Sum1/1 -> Mux/2
  [Pos_y_Offset_Arrow] -> Sum1/1
  Mux3/1 -> Scaling_L_x/1
  Demux/1 -> Mux3/3
  Mux1/1 -> Scaling_L_y/1
  Mux2/1 -> Scaling_L_z/1
  [Scaling_Fxy_Arrow] -> Mux2/2, Mux2/1, Mux1/2, Mux1/1, Mux3/2, Mux3/1
  Demux/3 -> Mux2/3
  Product2/1 -> Demux/1
  VehicleDynamics_Animation/1 -> Bus Selector1/1
  Bus Selector1/2 -> Sum/2  "<r_Dyn_RL_Tire[m]>"
  Sum/1 -> Mux/3
  Demux2/3 -> Sum/1
  Demux2/2 -> Sum1/2
  Demux2/1 -> Mux/1
  Bus Selector1/1 -> Demux2/1  "<Pos_RL_Wheel[x;y;z][m]>"
  Bus Selector1/3 -> Product2/1  "<F_RL_Tire_CoorSys_V[x;y;z][N]>"
  [Scaling_F_Tire] -> Product2/2
  [Pos_z_Offset_Arrow] -> Sum/3
  Mux/1 -> Translation_L/1

== system ASM_Traffic_A11/AnimationInterface/ANIMATION_INTERFACE/ASM_Vehicle/TireForceRightFront ==
  VehicleDynamics_Animation : Inport
  Bus Selector1 : BusSelector  OutputSignals=Pos_FR_Wheel[x;y;z][m],r_Dyn_FR_Tire[m],F_FR_Tire_CoorSys_V[x;y;z][N]
  Demux : Demux  Outputs=3
  Demux2 : Demux  Outputs=3
      settings: DisplayOption=none
  Mux{,1..3} (4 alike) : Mux  Inputs=3
  Product2 : Product  SaturateOnIntegerOverflow=on  OutDataTypeStr=Inherit: Same as first input
  Sum : Sum  Inputs=+-+  InputSameDT=on  SaturateOnIntegerOverflow=on  OutDataTypeStr=Inherit: Same as first input
  Sum1 : Sum  Inputs=-+  InputSameDT=on  SaturateOnIntegerOverflow=on  OutDataTypeStr=Inherit: Same as first input
  Translation_R : Outport  VectorParamsAs1DForOutWhenUnconnected=off
  Scaling_R_x : Outport  Port=2  VectorParamsAs1DForOutWhenUnconnected=off
  Scaling_R_y : Outport  Port=3  VectorParamsAs1DForOutWhenUnconnected=off
  Scaling_R_z : Outport  Port=4  VectorParamsAs1DForOutWhenUnconnected=off
  wires:
  Demux/2 -> Mux1/3
  Sum1/1 -> Mux/2
  [Pos_y_Offset_Arrow] -> Sum1/1
  Mux3/1 -> Scaling_R_x/1
  Demux/1 -> Mux3/3
  Mux1/1 -> Scaling_R_y/1
  Mux2/1 -> Scaling_R_z/1
  [Scaling_Fxy_Arrow] -> Mux2/2, Mux2/1, Mux1/2, Mux1/1, Mux3/2, Mux3/1
  Demux/3 -> Mux2/3
  Product2/1 -> Demux/1
  VehicleDynamics_Animation/1 -> Bus Selector1/1
  Bus Selector1/2 -> Sum/2  "<r_Dyn_FR_Tire[m]>"
  Sum/1 -> Mux/3
  Demux2/3 -> Sum/1
  Demux2/2 -> Sum1/2
  Demux2/1 -> Mux/1
  Bus Selector1/1 -> Demux2/1  "<Pos_FR_Wheel[x;y;z][m]>"
  Bus Selector1/3 -> Product2/1  "<F_FR_Tire_CoorSys_V[x;y;z][N]>"
  [Scaling_F_Tire] -> Product2/2
  [Pos_z_Offset_Arrow] -> Sum/3
  Mux/1 -> Translation_R/1

== system ASM_Traffic_A11/AnimationInterface/ANIMATION_INTERFACE/ASM_Vehicle/TireForceRightRear ==
  VehicleDynamics_Animation : Inport
  Bus Selector1 : BusSelector  OutputSignals=Pos_RR_Wheel[x;y;z][m],r_Dyn_RR_Tire[m],F_RR_Tire_CoorSys_V[x;y;z][N]
  Demux : Demux  Outputs=3
  Demux2 : Demux  Outputs=3
      settings: DisplayOption=none
  Mux{,1..3} (4 alike) : Mux  Inputs=3
  Product2 : Product  SaturateOnIntegerOverflow=on  OutDataTypeStr=Inherit: Same as first input
  Sum : Sum  Inputs=+-+  InputSameDT=on  SaturateOnIntegerOverflow=on  OutDataTypeStr=Inherit: Same as first input
  Sum1 : Sum  Inputs=-+  InputSameDT=on  SaturateOnIntegerOverflow=on  OutDataTypeStr=Inherit: Same as first input
  Translation_R : Outport  VectorParamsAs1DForOutWhenUnconnected=off
  Scaling_R_x : Outport  Port=2  VectorParamsAs1DForOutWhenUnconnected=off
  Scaling_R_y : Outport  Port=3  VectorParamsAs1DForOutWhenUnconnected=off
  Scaling_R_z : Outport  Port=4  VectorParamsAs1DForOutWhenUnconnected=off
  wires:
  Demux/2 -> Mux1/3
  Sum1/1 -> Mux/2
  [Pos_y_Offset_Arrow] -> Sum1/1
  Mux3/1 -> Scaling_R_x/1
  Demux/1 -> Mux3/3
  Mux1/1 -> Scaling_R_y/1
  Mux2/1 -> Scaling_R_z/1
  [Scaling_Fxy_Arrow] -> Mux2/2, Mux2/1, Mux1/2, Mux1/1, Mux3/2, Mux3/1
  Demux/3 -> Mux2/3
  Product2/1 -> Demux/1
  VehicleDynamics_Animation/1 -> Bus Selector1/1
  Bus Selector1/2 -> Sum/2  "<r_Dyn_RR_Tire[m]>"
  Sum/1 -> Mux/3
  Demux2/3 -> Sum/1
  Demux2/2 -> Sum1/2
  Demux2/1 -> Mux/1
  Bus Selector1/1 -> Demux2/1  "<Pos_RR_Wheel[x;y;z][m]>"
  Bus Selector1/3 -> Product2/1  "<F_RR_Tire_CoorSys_V[x;y;z][N]>"
  [Scaling_F_Tire] -> Product2/2
  [Pos_z_Offset_Arrow] -> Sum/3
  Mux/1 -> Translation_R/1

== system ASM_Traffic_A11/AnimationInterface/ANIMATION_INTERFACE/ASM_Vehicle/Wheel_FL ==
  VehicleDynamics_Animation : Inport
  Bus Selector1 : BusSelector  OutputSignals=Pos_FL_Wheel[x;y;z][m],Angle_FL_Wheel[Toe;Camber][deg],Angle_Rot_FL_Wheel[deg],r_Dyn_FL_Tire[m],Const_r_unloaded_Tire_FL[m]
  Constant1 : Constant
  Divide : Product  Inputs=*/
  Multiport Switch : MultiPortSwitch  DataPortOrder=Zero-based contiguous  Inputs=2  zeroidx=on  SaturateOnIntegerOverflow=off  InputSameDT=off
  Mux4 : Mux  Inputs=3
  Mux7 : Mux  Inputs=2
  Rotation_WheelFL : Gain  Gain=[-1 -1 1]
  Translation : Outport
  Rotation : Outport  Port=2
  Scaling : Outport  Port=3
  wires:
  Multiport Switch/1 -> Divide/2
  Bus Selector1/5 -> Multiport Switch/2  "<Const_r_unloaded_Tire_FL[m]>"
  [Sw_TireRadius] -> Multiport Switch/1
  Divide/1 -> Mux4/1, Mux4/3
  [TireRadius] -> Multiport Switch/3
  Constant1/1 -> Mux4/2
  VehicleDynamics_Animation/1 -> Bus Selector1/1
  Bus Selector1/1 -> Translation/1  "<Pos_FL_Wheel[x;y;z][m]>"
  Bus Selector1/3 -> Mux7/2  "<Angle_Rot_FL_Wheel[deg]>"
  Bus Selector1/2 -> Mux7/1  "<Angle_FL_Wheel[Toe;Camber][deg]>"
  Bus Selector1/4 -> Divide/1  "<r_Dyn_FL_Tire[m]>"
  Mux4/1 -> Scaling/1
  Rotation_WheelFL/1 -> Rotation/1
  Mux7/1 -> Rotation_WheelFL/1

== system ASM_Traffic_A11/AnimationInterface/ANIMATION_INTERFACE/ASM_Vehicle/Wheel_FR ==
  VehicleDynamics_Animation : Inport
  Bus Selector1 : BusSelector  OutputSignals=Pos_FR_Wheel[x;y;z][m],Angle_FR_Wheel[Toe;Camber][deg],Angle_Rot_FR_Wheel[deg],r_Dyn_FR_Tire[m],Const_r_unloaded_Tire_FR[m]
  Constant1 : Constant
  Divide : Product  Inputs=*/
  Multiport Switch : MultiPortSwitch  DataPortOrder=Zero-based contiguous  Inputs=2  zeroidx=on  SaturateOnIntegerOverflow=off  InputSameDT=off
  Mux4 : Mux  Inputs=3
  Mux7 : Mux  Inputs=2
  Rotation_WheelFR : Gain  Gain=[1 1 1]
  Translation : Outport
  Rotation : Outport  Port=2
  Scaling : Outport  Port=3
  wires:
  [Sw_TireRadius] -> Multiport Switch/1
  Bus Selector1/5 -> Multiport Switch/2  "<Const_r_unloaded_Tire_FR[m]>"
  [TireRadius] -> Multiport Switch/3
  Multiport Switch/1 -> Divide/2
  Mux7/1 -> Rotation_WheelFR/1
  Rotation_WheelFR/1 -> Rotation/1
  Mux4/1 -> Scaling/1
  Bus Selector1/4 -> Divide/1  "<r_Dyn_FR_Tire[m]>"
  Bus Selector1/2 -> Mux7/1  "<Angle_FR_Wheel[Toe;Camber][deg]>"
  Bus Selector1/3 -> Mux7/2  "<Angle_Rot_FR_Wheel[deg]>"
  Bus Selector1/1 -> Translation/1  "<Pos_FR_Wheel[x;y;z][m]>"
  VehicleDynamics_Animation/1 -> Bus Selector1/1
  Constant1/1 -> Mux4/2
  Divide/1 -> Mux4/3, Mux4/1

== system ASM_Traffic_A11/AnimationInterface/ANIMATION_INTERFACE/ASM_Vehicle/Wheel_RL ==
  VehicleDynamics_Animation : Inport
  Bus Selector1 : BusSelector  OutputSignals=Pos_RL_Wheel[x;y;z][m],Angle_RL_Wheel[Toe;Camber][deg],Angle_Rot_RL_Wheel[deg],r_Dyn_RL_Tire[m],Const_r_unloaded_Tire_RL[m]
  Constant1 : Constant
  Divide : Product  Inputs=*/
  Multiport Switch : MultiPortSwitch  DataPortOrder=Zero-based contiguous  Inputs=2  zeroidx=on  SaturateOnIntegerOverflow=off  InputSameDT=off
  Mux4 : Mux  Inputs=3
  Mux7 : Mux  Inputs=2
  Rotation_WheelRL : Gain  Gain=[-1 -1 1]
  Translation : Outport
  Rotation : Outport  Port=2
  Scaling : Outport  Port=3
  wires:
  [Sw_TireRadius] -> Multiport Switch/1
  Bus Selector1/5 -> Multiport Switch/2  "<Const_r_unloaded_Tire_RL[m]>"
  [TireRadius] -> Multiport Switch/3
  Multiport Switch/1 -> Divide/2
  Mux7/1 -> Rotation_WheelRL/1
  Rotation_WheelRL/1 -> Rotation/1
  Mux4/1 -> Scaling/1
  Bus Selector1/4 -> Divide/1  "<r_Dyn_RL_Tire[m]>"
  Bus Selector1/2 -> Mux7/1  "<Angle_RL_Wheel[Toe;Camber][deg]>"
  Bus Selector1/3 -> Mux7/2  "<Angle_Rot_RL_Wheel[deg]>"
  Bus Selector1/1 -> Translation/1  "<Pos_RL_Wheel[x;y;z][m]>"
  VehicleDynamics_Animation/1 -> Bus Selector1/1
  Constant1/1 -> Mux4/2
  Divide/1 -> Mux4/3, Mux4/1

== system ASM_Traffic_A11/AnimationInterface/ANIMATION_INTERFACE/ASM_Vehicle/Wheel_RR ==
  VehicleDynamics_Animation : Inport
  Bus Selector5 : BusSelector  OutputSignals=Pos_RR_Wheel[x;y;z][m],Angle_RR_Wheel[Toe;Camber][deg],Angle_Rot_RR_Wheel[deg],r_Dyn_RR_Tire[m],Const_r_unloaded_Tire_RR[m]
  Constant1 : Constant
  Divide : Product  Inputs=*/
  Multiport Switch : MultiPortSwitch  DataPortOrder=Zero-based contiguous  Inputs=2  zeroidx=on  SaturateOnIntegerOverflow=off  InputSameDT=off
  Mux4 : Mux  Inputs=3
  Mux7 : Mux  Inputs=2
  Rotation_WheelRR : Gain  Gain=[1 1 1]
  Translation : Outport
  Rotation : Outport  Port=2
  Scaling : Outport  Port=3
  wires:
  [Sw_TireRadius] -> Multiport Switch/1
  Bus Selector5/5 -> Multiport Switch/2  "<Const_r_unloaded_Tire_RR[m]>"
  [TireRadius] -> Multiport Switch/3
  Multiport Switch/1 -> Divide/2
  Divide/1 -> Mux4/1, Mux4/3
  Constant1/1 -> Mux4/2
  VehicleDynamics_Animation/1 -> Bus Selector5/1
  Bus Selector5/1 -> Translation/1  "<Pos_RR_Wheel[x;y;z][m]>"
  Bus Selector5/3 -> Mux7/2  "<Angle_Rot_RR_Wheel[deg]>"
  Bus Selector5/2 -> Mux7/1  "<Angle_RR_Wheel[Toe;Camber][deg]>"
  Bus Selector5/4 -> Divide/1  "<r_Dyn_RR_Tire[m]>"
  Mux4/1 -> Scaling/1
  Rotation_WheelRR/1 -> Rotation/1
  Mux7/1 -> Rotation_WheelRR/1

== system ASM_Traffic_A11/AnimationInterface/ANIMATION_INTERFACE/Bounding_Boxes/BoundingBox_1 ==
  Index[] : Inport
  BoundigBoxes_Animation : Inport  Port=2
  Bus Selector : BusSelector  OutputSignals=Pos_x_CoorSysE[m],Pos_y_CoorSysE[m],Pos_z_CoorSysE[m],Angle_z_Objects_CoorSysE[deg],Angle_y_Objects_CoorSysE[deg],Angle_x_Objects_CoorSysE[deg],Length_Object[m],Width_Object[m],Height_Object[m]
  Mux : Mux  Inputs=3
  Mux1 : Mux  Inputs=3
  Mux2 : Mux  Inputs=3
  Selector{1..9} (9 alike) : Selector  IndexOptions=Index vector (port)  Indices=[1 3]  OutputSizes=1
  Pos_CoorSysE[m] : Outport  VectorParamsAs1DForOutWhenUnconnected=off
  Angle_CoorSysE[m] : Outport  Port=2  VectorParamsAs1DForOutWhenUnconnected=off
  Dimensions[m] : Outport  Port=3  VectorParamsAs1DForOutWhenUnconnected=off
  wires:
  Bus Selector/9 -> Selector9/1  "<Height_Object[m]>"
  Bus Selector/8 -> Selector8/1  "<Width_Object[m]>"
  Bus Selector/7 -> Selector6/1  "<Length_Object[m]>"
  Bus Selector/6 -> Selector7/1  "<Angle_x_Objects_CoorSysE[deg]>"
  Bus Selector/5 -> Selector5/1  "<Angle_y_Objects_CoorSysE[deg]>"
  Bus Selector/4 -> Selector4/1  "<Angle_z_Objects_CoorSysE[deg]>"
  Bus Selector/3 -> Selector3/1  "<Pos_z_CoorSysE[m]>"
  Bus Selector/2 -> Selector2/1  "<Pos_y_CoorSysE[m]>"
  Bus Selector/1 -> Selector1/1  "<Pos_x_CoorSysE[m]>"
  BoundigBoxes_Animation/1 -> Bus Selector/1
  Selector5/1 -> Mux1/2
  Mux1/1 -> Angle_CoorSysE[m]/1
  Mux/1 -> Pos_CoorSysE[m]/1
  Index[]/1 -> Selector3/2, Selector4/2, Selector9/2, Selector8/2, Selector6/2, Selector7/2, Selector5/2, Selector2/2, Selector1/2
  Selector1/1 -> Mux/1
  Selector2/1 -> Mux/2
  Selector3/1 -> Mux/3
  Selector7/1 -> Mux1/3
  Selector4/1 -> Mux1/1
  Selector6/1 -> Mux2/1
  Selector8/1 -> Mux2/2
  Selector9/1 -> Mux2/3
  Mux2/1 -> Dimensions[m]/1

== system ASM_Traffic_A11/AnimationInterface/ANIMATION_INTERFACE/Bounding_Boxes/BoundingBox_10 ==
  Index[] : Inport
  BoundigBoxes_Animation : Inport  Port=2
  Bus Selector : BusSelector  OutputSignals=Pos_x_CoorSysE[m],Pos_y_CoorSysE[m],Pos_z_CoorSysE[m],Angle_z_Objects_CoorSysE[deg],Angle_y_Objects_CoorSysE[deg],Angle_x_Objects_CoorSysE[deg],Length_Object[m],Width_Object[m],Height_Object[m]
  Mux : Mux  Inputs=3
  Mux1 : Mux  Inputs=3
  Mux2 : Mux  Inputs=3
  Selector{1..9} (9 alike) : Selector  IndexOptions=Index vector (port)  Indices=[1 3]  OutputSizes=1
  Pos_CoorSysE[m] : Outport  VectorParamsAs1DForOutWhenUnconnected=off
  Angle_CoorSysE[m] : Outport  Port=2  VectorParamsAs1DForOutWhenUnconnected=off
  Dimensions[m] : Outport  Port=3  VectorParamsAs1DForOutWhenUnconnected=off
  wires:
  Bus Selector/9 -> Selector9/1  "<Height_Object[m]>"
  Bus Selector/8 -> Selector8/1  "<Width_Object[m]>"
  Bus Selector/7 -> Selector6/1  "<Length_Object[m]>"
  Bus Selector/6 -> Selector7/1  "<Angle_x_Objects_CoorSysE[deg]>"
  Bus Selector/5 -> Selector5/1  "<Angle_y_Objects_CoorSysE[deg]>"
  Bus Selector/4 -> Selector4/1  "<Angle_z_Objects_CoorSysE[deg]>"
  Bus Selector/3 -> Selector3/1  "<Pos_z_CoorSysE[m]>"
  Bus Selector/2 -> Selector2/1  "<Pos_y_CoorSysE[m]>"
  Bus Selector/1 -> Selector1/1  "<Pos_x_CoorSysE[m]>"
  BoundigBoxes_Animation/1 -> Bus Selector/1
  Selector5/1 -> Mux1/2
  Mux1/1 -> Angle_CoorSysE[m]/1
  Mux/1 -> Pos_CoorSysE[m]/1
  Index[]/1 -> Selector3/2, Selector4/2, Selector9/2, Selector8/2, Selector6/2, Selector7/2, Selector5/2, Selector2/2, Selector1/2
  Selector1/1 -> Mux/1
  Selector2/1 -> Mux/2
  Selector3/1 -> Mux/3
  Selector7/1 -> Mux1/3
  Selector4/1 -> Mux1/1
  Selector6/1 -> Mux2/1
  Selector8/1 -> Mux2/2
  Selector9/1 -> Mux2/3
  Mux2/1 -> Dimensions[m]/1

== system ASM_Traffic_A11/AnimationInterface/ANIMATION_INTERFACE/Bounding_Boxes/BoundingBox_2 ==
  Index[] : Inport
  BoundigBoxes_Animation : Inport  Port=2
  Bus Selector : BusSelector  OutputSignals=Pos_x_CoorSysE[m],Pos_y_CoorSysE[m],Pos_z_CoorSysE[m],Angle_z_Objects_CoorSysE[deg],Angle_y_Objects_CoorSysE[deg],Angle_x_Objects_CoorSysE[deg],Length_Object[m],Width_Object[m],Height_Object[m]
  Mux : Mux  Inputs=3
  Mux1 : Mux  Inputs=3
  Mux2 : Mux  Inputs=3
  Selector{1..9} (9 alike) : Selector  IndexOptions=Index vector (port)  Indices=[1 3]  OutputSizes=1
  Pos_CoorSysE[m] : Outport  VectorParamsAs1DForOutWhenUnconnected=off
  Angle_CoorSysE[m] : Outport  Port=2  VectorParamsAs1DForOutWhenUnconnected=off
  Dimensions[m] : Outport  Port=3  VectorParamsAs1DForOutWhenUnconnected=off
  wires:
  Mux2/1 -> Dimensions[m]/1
  Selector9/1 -> Mux2/3
  Selector8/1 -> Mux2/2
  Selector6/1 -> Mux2/1
  Selector4/1 -> Mux1/1
  Selector7/1 -> Mux1/3
  Selector3/1 -> Mux/3
  Selector2/1 -> Mux/2
  Selector1/1 -> Mux/1
  Index[]/1 -> Selector1/2, Selector2/2, Selector5/2, Selector7/2, Selector6/2, Selector8/2, Selector9/2, Selector4/2, Selector3/2
  Mux/1 -> Pos_CoorSysE[m]/1
  Mux1/1 -> Angle_CoorSysE[m]/1
  Selector5/1 -> Mux1/2
  BoundigBoxes_Animation/1 -> Bus Selector/1
  Bus Selector/1 -> Selector1/1  "<Pos_x_CoorSysE[m]>"
  Bus Selector/2 -> Selector2/1  "<Pos_y_CoorSysE[m]>"
  Bus Selector/3 -> Selector3/1  "<Pos_z_CoorSysE[m]>"
  Bus Selector/4 -> Selector4/1  "<Angle_z_Objects_CoorSysE[deg]>"
  Bus Selector/5 -> Selector5/1  "<Angle_y_Objects_CoorSysE[deg]>"
  Bus Selector/6 -> Selector7/1  "<Angle_x_Objects_CoorSysE[deg]>"
  Bus Selector/7 -> Selector6/1  "<Length_Object[m]>"
  Bus Selector/8 -> Selector8/1  "<Width_Object[m]>"
  Bus Selector/9 -> Selector9/1  "<Height_Object[m]>"

== system ASM_Traffic_A11/AnimationInterface/ANIMATION_INTERFACE/Bounding_Boxes/BoundingBox_3 ==
  Index[] : Inport
  BoundigBoxes_Animation : Inport  Port=2
  Bus Selector : BusSelector  OutputSignals=Pos_x_CoorSysE[m],Pos_y_CoorSysE[m],Pos_z_CoorSysE[m],Angle_z_Objects_CoorSysE[deg],Angle_y_Objects_CoorSysE[deg],Angle_x_Objects_CoorSysE[deg],Length_Object[m],Width_Object[m],Height_Object[m]
  Mux : Mux  Inputs=3
  Mux1 : Mux  Inputs=3
  Mux2 : Mux  Inputs=3
  Selector{1..9} (9 alike) : Selector  IndexOptions=Index vector (port)  Indices=[1 3]  OutputSizes=1
  Pos_CoorSysE[m] : Outport  VectorParamsAs1DForOutWhenUnconnected=off
  Angle_CoorSysE[m] : Outport  Port=2  VectorParamsAs1DForOutWhenUnconnected=off
  Dimensions[m] : Outport  Port=3  VectorParamsAs1DForOutWhenUnconnected=off
  wires:
  Mux2/1 -> Dimensions[m]/1
  Selector9/1 -> Mux2/3
  Selector8/1 -> Mux2/2
  Selector6/1 -> Mux2/1
  Selector4/1 -> Mux1/1
  Selector7/1 -> Mux1/3
  Selector3/1 -> Mux/3
  Selector2/1 -> Mux/2
  Selector1/1 -> Mux/1
  Index[]/1 -> Selector1/2, Selector2/2, Selector5/2, Selector7/2, Selector6/2, Selector8/2, Selector9/2, Selector4/2, Selector3/2
  Mux/1 -> Pos_CoorSysE[m]/1
  Mux1/1 -> Angle_CoorSysE[m]/1
  Selector5/1 -> Mux1/2
  BoundigBoxes_Animation/1 -> Bus Selector/1
  Bus Selector/1 -> Selector1/1  "<Pos_x_CoorSysE[m]>"
  Bus Selector/2 -> Selector2/1  "<Pos_y_CoorSysE[m]>"
  Bus Selector/3 -> Selector3/1  "<Pos_z_CoorSysE[m]>"
  Bus Selector/4 -> Selector4/1  "<Angle_z_Objects_CoorSysE[deg]>"
  Bus Selector/5 -> Selector5/1  "<Angle_y_Objects_CoorSysE[deg]>"
  Bus Selector/6 -> Selector7/1  "<Angle_x_Objects_CoorSysE[deg]>"
  Bus Selector/7 -> Selector6/1  "<Length_Object[m]>"
  Bus Selector/8 -> Selector8/1  "<Width_Object[m]>"
  Bus Selector/9 -> Selector9/1  "<Height_Object[m]>"
